simulink model "ASM_AnimationInterface"  (R2024a)
settings: Solver=ode1  StartTime=SIM.tstart.v  StopTime=SIM.tend.v  FixedStep=SIM.StepSize.v  RelTol=1e-3
PostLoadFcn:
  | , if any(exist('dsrtsu_mdlpostloadfcn', 'file') ~= 0), dsrtsu_mdlpostloadfcn('Execute', bdroot); end,
undefined symbols (not defined in the file): a0b2, b98103fe8ad365046cd0, dsmsi, MDL, SIM
libraries: simulink x22, dsmsilib x15, dsmpblib x4, ASM_Environment_lib x1
(part 6 of 7)

== system ASM_AnimationInterface/AnimationInterface/ANIMATION_INTERFACE/ASM_Vehicle/TireForceLeftFront ==
  VehicleDynamics_Animation : Inport
  Bus Selector1 : BusSelector  OutputSignals=Pos_FL_Wheel[x;y;z][m],r_Dyn_FL_Tire[m],F_FL_Tire_CoorSys_V[x;y;z][N]
  Demux : Demux  Outputs=3
  Demux2 : Demux  Outputs=3
      settings: DisplayOption=none
  Mux{,1..3} (4 alike) : Mux  Inputs=3
  Product2 : Product  SaturateOnIntegerOverflow=on  OutDataTypeStr=Inherit: Same as first input
  Sum : Sum  Inputs=+-+  InputSameDT=on  SaturateOnIntegerOverflow=on  OutDataTypeStr=Inherit: Same as first input
  Sum1 : Sum  InputSameDT=on  SaturateOnIntegerOverflow=on  OutDataTypeStr=Inherit: Same as first input
  Translation_L : Outport  VectorParamsAs1DForOutWhenUnconnected=off
  Scaling_L_x : Outport  Port=2  VectorParamsAs1DForOutWhenUnconnected=off
  Scaling_L_y : Outport  Port=3  VectorParamsAs1DForOutWhenUnconnected=off
  Scaling_L_z : Outport  Port=4  VectorParamsAs1DForOutWhenUnconnected=off
  wires:
  Mux/1 -> Translation_L/1
  [Pos_z_Offset_Arrow] -> Sum/3
  [Scaling_F_Tire] -> Product2/2
  Bus Selector1/3 -> Product2/1  "<F_FL_Tire_CoorSys_V[x;y;z][N]>"
  Bus Selector1/1 -> Demux2/1  "<Pos_FL_Wheel[x;y;z][m]>"
  Demux2/1 -> Mux/1
  Demux2/2 -> Sum1/2
  Demux2/3 -> Sum/1
  Sum/1 -> Mux/3
  Bus Selector1/2 -> Sum/2  "<r_Dyn_FL_Tire[m]>"
  VehicleDynamics_Animation/1 -> Bus Selector1/1
  Product2/1 -> Demux/1
  [Scaling_Fxy_Arrow] -> Mux3/1, Mux3/2, Mux1/1, Mux1/2, Mux2/1, Mux2/2
  Mux2/1 -> Scaling_L_z/1
  Mux1/1 -> Scaling_L_y/1
  Demux/1 -> Mux3/3
  Mux3/1 -> Scaling_L_x/1
  [Pos_y_Offset_Arrow] -> Sum1/1
  Sum1/1 -> Mux/2
  Demux/3 -> Mux2/3
  Demux/2 -> Mux1/3

== system ASM_AnimationInterface/AnimationInterface/ANIMATION_INTERFACE/ASM_Vehicle/TireForceLeftRear ==
  VehicleDynamics_Animation : Inport
  Bus Selector1 : BusSelector  OutputSignals=Pos_RL_Wheel[x;y;z][m],r_Dyn_RL_Tire[m],F_RL_Tire_CoorSys_V[x;y;z][N]
  Demux : Demux  Outputs=3
  Demux2 : Demux  Outputs=3
      settings: DisplayOption=none
  Mux{,1..3} (4 alike) : Mux  Inputs=3
  Product2 : Product  SaturateOnIntegerOverflow=on  OutDataTypeStr=Inherit: Same as first input
  Sum : Sum  Inputs=+-+  InputSameDT=on  SaturateOnIntegerOverflow=on  OutDataTypeStr=Inherit: Same as first input
  Sum1 : Sum  InputSameDT=on  SaturateOnIntegerOverflow=on  OutDataTypeStr=Inherit: Same as first input
  Translation_L : Outport  VectorParamsAs1DForOutWhenUnconnected=off
  Scaling_L_x : Outport  Port=2  VectorParamsAs1DForOutWhenUnconnected=off
  Scaling_L_y : Outport  Port=3  VectorParamsAs1DForOutWhenUnconnected=off
  Scaling_L_z : Outport  Port=4  VectorParamsAs1DForOutWhenUnconnected=off
  wires:
  Mux/1 -> Translation_L/1
  [Pos_z_Offset_Arrow] -> Sum/3
  [Scaling_F_Tire] -> Product2/2
  Bus Selector1/3 -> Product2/1  "<F_RL_Tire_CoorSys_V[x;y;z][N]>"
  Bus Selector1/1 -> Demux2/1  "<Pos_RL_Wheel[x;y;z][m]>"
  Demux2/1 -> Mux/1
  Demux2/2 -> Sum1/2
  Demux2/3 -> Sum/1
  Sum/1 -> Mux/3
  Bus Selector1/2 -> Sum/2  "<r_Dyn_RL_Tire[m]>"
  VehicleDynamics_Animation/1 -> Bus Selector1/1
  Product2/1 -> Demux/1
  Demux/3 -> Mux2/3
  [Scaling_Fxy_Arrow] -> Mux3/1, Mux3/2, Mux1/1, Mux1/2, Mux2/1, Mux2/2
  Mux2/1 -> Scaling_L_z/1
  Mux1/1 -> Scaling_L_y/1
  Demux/1 -> Mux3/3
  Mux3/1 -> Scaling_L_x/1
  [Pos_y_Offset_Arrow] -> Sum1/1
  Sum1/1 -> Mux/2
  Demux/2 -> Mux1/3

== system ASM_AnimationInterface/AnimationInterface/ANIMATION_INTERFACE/ASM_Vehicle/TireForceRightFront ==
  VehicleDynamics_Animation : Inport
  Bus Selector1 : BusSelector  OutputSignals=Pos_FR_Wheel[x;y;z][m],r_Dyn_FR_Tire[m],F_FR_Tire_CoorSys_V[x;y;z][N]
  Demux : Demux  Outputs=3
  Demux2 : Demux  Outputs=3
      settings: DisplayOption=none
  Mux{,1..3} (4 alike) : Mux  Inputs=3
  Product2 : Product  SaturateOnIntegerOverflow=on  OutDataTypeStr=Inherit: Same as first input
  Sum : Sum  Inputs=+-+  InputSameDT=on  SaturateOnIntegerOverflow=on  OutDataTypeStr=Inherit: Same as first input
  Sum1 : Sum  Inputs=-+  InputSameDT=on  SaturateOnIntegerOverflow=on  OutDataTypeStr=Inherit: Same as first input
  Translation_R : Outport  VectorParamsAs1DForOutWhenUnconnected=off
  Scaling_R_x : Outport  Port=2  VectorParamsAs1DForOutWhenUnconnected=off
  Scaling_R_y : Outport  Port=3  VectorParamsAs1DForOutWhenUnconnected=off
  Scaling_R_z : Outport  Port=4  VectorParamsAs1DForOutWhenUnconnected=off
  wires:
  Mux/1 -> Translation_R/1
  [Pos_z_Offset_Arrow] -> Sum/3
  [Scaling_F_Tire] -> Product2/2
  Bus Selector1/3 -> Product2/1  "<F_FR_Tire_CoorSys_V[x;y;z][N]>"
  Bus Selector1/1 -> Demux2/1  "<Pos_FR_Wheel[x;y;z][m]>"
  Demux2/1 -> Mux/1
  Demux2/2 -> Sum1/2
  Demux2/3 -> Sum/1
  Sum/1 -> Mux/3
  Bus Selector1/2 -> Sum/2  "<r_Dyn_FR_Tire[m]>"
  VehicleDynamics_Animation/1 -> Bus Selector1/1
  Product2/1 -> Demux/1
  Demux/3 -> Mux2/3
  [Scaling_Fxy_Arrow] -> Mux3/1, Mux3/2, Mux1/1, Mux1/2, Mux2/1, Mux2/2
  Mux2/1 -> Scaling_R_z/1
  Mux1/1 -> Scaling_R_y/1
  Demux/1 -> Mux3/3
  Mux3/1 -> Scaling_R_x/1
  [Pos_y_Offset_Arrow] -> Sum1/1
  Sum1/1 -> Mux/2
  Demux/2 -> Mux1/3

== system ASM_AnimationInterface/AnimationInterface/ANIMATION_INTERFACE/ASM_Vehicle/TireForceRightRear ==
  VehicleDynamics_Animation : Inport
  Bus Selector1 : BusSelector  OutputSignals=Pos_RR_Wheel[x;y;z][m],r_Dyn_RR_Tire[m],F_RR_Tire_CoorSys_V[x;y;z][N]
  Demux : Demux  Outputs=3
  Demux2 : Demux  Outputs=3
      settings: DisplayOption=none
  Mux{,1..3} (4 alike) : Mux  Inputs=3
  Product2 : Product  SaturateOnIntegerOverflow=on  OutDataTypeStr=Inherit: Same as first input
  Sum : Sum  Inputs=+-+  InputSameDT=on  SaturateOnIntegerOverflow=on  OutDataTypeStr=Inherit: Same as first input
  Sum1 : Sum  Inputs=-+  InputSameDT=on  SaturateOnIntegerOverflow=on  OutDataTypeStr=Inherit: Same as first input
  Translation_R : Outport  VectorParamsAs1DForOutWhenUnconnected=off
  Scaling_R_x : Outport  Port=2  VectorParamsAs1DForOutWhenUnconnected=off
  Scaling_R_y : Outport  Port=3  VectorParamsAs1DForOutWhenUnconnected=off
  Scaling_R_z : Outport  Port=4  VectorParamsAs1DForOutWhenUnconnected=off
  wires:
  Mux/1 -> Translation_R/1
  [Pos_z_Offset_Arrow] -> Sum/3
  [Scaling_F_Tire] -> Product2/2
  Bus Selector1/3 -> Product2/1  "<F_RR_Tire_CoorSys_V[x;y;z][N]>"
  Bus Selector1/1 -> Demux2/1  "<Pos_RR_Wheel[x;y;z][m]>"
  Demux2/1 -> Mux/1
  Demux2/2 -> Sum1/2
  Demux2/3 -> Sum/1
  Sum/1 -> Mux/3
  Bus Selector1/2 -> Sum/2  "<r_Dyn_RR_Tire[m]>"
  VehicleDynamics_Animation/1 -> Bus Selector1/1
  Product2/1 -> Demux/1
  Demux/3 -> Mux2/3
  [Scaling_Fxy_Arrow] -> Mux3/1, Mux3/2, Mux1/1, Mux1/2, Mux2/1, Mux2/2
  Mux2/1 -> Scaling_R_z/1
  Mux1/1 -> Scaling_R_y/1
  Demux/1 -> Mux3/3
  Mux3/1 -> Scaling_R_x/1
  [Pos_y_Offset_Arrow] -> Sum1/1
  Sum1/1 -> Mux/2
  Demux/2 -> Mux1/3

== system ASM_AnimationInterface/AnimationInterface/ANIMATION_INTERFACE/ASM_Vehicle/Wheel_FL ==
  VehicleDynamics_Animation : Inport
  Bus Selector1 : BusSelector  OutputSignals=Pos_FL_Wheel[x;y;z][m],Angle_FL_Wheel[Toe;Camber][deg],Angle_Rot_FL_Wheel[deg],r_Dyn_FL_Tire[m],Const_r_unloaded_Tire_FL[m]
  Constant1 : Constant
  Divide : Product  Inputs=*/
  Multiport Switch : MultiPortSwitch  DataPortOrder=Zero-based contiguous  Inputs=2  zeroidx=on  SaturateOnIntegerOverflow=off  InputSameDT=off
  Mux4 : Mux  Inputs=3
  Mux7 : Mux  Inputs=2
  Rotation_WheelFL : Gain  Gain=[-1 -1 1]
  Translation : Outport
  Rotation : Outport  Port=2
  Scaling : Outport  Port=3
  wires:
  Mux7/1 -> Rotation_WheelFL/1
  Rotation_WheelFL/1 -> Rotation/1
  Mux4/1 -> Scaling/1
  Bus Selector1/4 -> Divide/1  "<r_Dyn_FL_Tire[m]>"
  Bus Selector1/2 -> Mux7/1  "<Angle_FL_Wheel[Toe;Camber][deg]>"
  Bus Selector1/3 -> Mux7/2  "<Angle_Rot_FL_Wheel[deg]>"
  Bus Selector1/1 -> Translation/1  "<Pos_FL_Wheel[x;y;z][m]>"
  VehicleDynamics_Animation/1 -> Bus Selector1/1
  Constant1/1 -> Mux4/2
  [TireRadius] -> Multiport Switch/3
  Divide/1 -> Mux4/3, Mux4/1
  [Sw_TireRadius] -> Multiport Switch/1
  Bus Selector1/5 -> Multiport Switch/2  "<Const_r_unloaded_Tire_FL[m]>"
  Multiport Switch/1 -> Divide/2

== system ASM_AnimationInterface/AnimationInterface/ANIMATION_INTERFACE/ASM_Vehicle/Wheel_FR ==
  VehicleDynamics_Animation : Inport
  Bus Selector1 : BusSelector  OutputSignals=Pos_FR_Wheel[x;y;z][m],Angle_FR_Wheel[Toe;Camber][deg],Angle_Rot_FR_Wheel[deg],r_Dyn_FR_Tire[m],Const_r_unloaded_Tire_FR[m]
  Constant1 : Constant
  Divide : Product  Inputs=*/
  Multiport Switch : MultiPortSwitch  DataPortOrder=Zero-based contiguous  Inputs=2  zeroidx=on  SaturateOnIntegerOverflow=off  InputSameDT=off
  Mux4 : Mux  Inputs=3
  Mux7 : Mux  Inputs=2
  Rotation_WheelFR : Gain  Gain=[1 1 1]
  Translation : Outport
  Rotation : Outport  Port=2
  Scaling : Outport  Port=3
  wires:
  Divide/1 -> Mux4/1, Mux4/3
  Constant1/1 -> Mux4/2
  VehicleDynamics_Animation/1 -> Bus Selector1/1
  Bus Selector1/1 -> Translation/1  "<Pos_FR_Wheel[x;y;z][m]>"
  Bus Selector1/3 -> Mux7/2  "<Angle_Rot_FR_Wheel[deg]>"
  Bus Selector1/2 -> Mux7/1  "<Angle_FR_Wheel[Toe;Camber][deg]>"
  Bus Selector1/4 -> Divide/1  "<r_Dyn_FR_Tire[m]>"
  Mux4/1 -> Scaling/1
  Rotation_WheelFR/1 -> Rotation/1
  Mux7/1 -> Rotation_WheelFR/1
  Multiport Switch/1 -> Divide/2
  [TireRadius] -> Multiport Switch/3
  Bus Selector1/5 -> Multiport Switch/2  "<Const_r_unloaded_Tire_FR[m]>"
  [Sw_TireRadius] -> Multiport Switch/1

== system ASM_AnimationInterface/AnimationInterface/ANIMATION_INTERFACE/ASM_Vehicle/Wheel_RL ==
  VehicleDynamics_Animation : Inport
  Bus Selector1 : BusSelector  OutputSignals=Pos_RL_Wheel[x;y;z][m],Angle_RL_Wheel[Toe;Camber][deg],Angle_Rot_RL_Wheel[deg],r_Dyn_RL_Tire[m],Const_r_unloaded_Tire_RL[m]
  Constant1 : Constant
  Divide : Product  Inputs=*/
  Multiport Switch : MultiPortSwitch  DataPortOrder=Zero-based contiguous  Inputs=2  zeroidx=on  SaturateOnIntegerOverflow=off  InputSameDT=off
  Mux4 : Mux  Inputs=3
  Mux7 : Mux  Inputs=2
  Rotation_WheelRL : Gain  Gain=[-1 -1 1]
  Translation : Outport
  Rotation : Outport  Port=2
  Scaling : Outport  Port=3
  wires:
  Divide/1 -> Mux4/1, Mux4/3
  Constant1/1 -> Mux4/2
  VehicleDynamics_Animation/1 -> Bus Selector1/1
  Bus Selector1/1 -> Translation/1  "<Pos_RL_Wheel[x;y;z][m]>"
  Bus Selector1/3 -> Mux7/2  "<Angle_Rot_RL_Wheel[deg]>"
  Bus Selector1/2 -> Mux7/1  "<Angle_RL_Wheel[Toe;Camber][deg]>"
  Bus Selector1/4 -> Divide/1  "<r_Dyn_RL_Tire[m]>"
  Mux4/1 -> Scaling/1
  Rotation_WheelRL/1 -> Rotation/1
  Mux7/1 -> Rotation_WheelRL/1
  Multiport Switch/1 -> Divide/2
  [TireRadius] -> Multiport Switch/3
  Bus Selector1/5 -> Multiport Switch/2  "<Const_r_unloaded_Tire_RL[m]>"
  [Sw_TireRadius] -> Multiport Switch/1

== system ASM_AnimationInterface/AnimationInterface/ANIMATION_INTERFACE/ASM_Vehicle/Wheel_RR ==
  VehicleDynamics_Animation : Inport
  Bus Selector5 : BusSelector  OutputSignals=Pos_RR_Wheel[x;y;z][m],Angle_RR_Wheel[Toe;Camber][deg],Angle_Rot_RR_Wheel[deg],r_Dyn_RR_Tire[m],Const_r_unloaded_Tire_RR[m]
  Constant1 : Constant
  Divide : Product  Inputs=*/
  Multiport Switch : MultiPortSwitch  DataPortOrder=Zero-based contiguous  Inputs=2  zeroidx=on  SaturateOnIntegerOverflow=off  InputSameDT=off
  Mux4 : Mux  Inputs=3
  Mux7 : Mux  Inputs=2
  Rotation_WheelRR : Gain  Gain=[1 1 1]
  Translation : Outport
  Rotation : Outport  Port=2
  Scaling : Outport  Port=3
  wires:
  Mux7/1 -> Rotation_WheelRR/1
  Rotation_WheelRR/1 -> Rotation/1
  Mux4/1 -> Scaling/1
  Bus Selector5/4 -> Divide/1  "<r_Dyn_RR_Tire[m]>"
  Bus Selector5/2 -> Mux7/1  "<Angle_RR_Wheel[Toe;Camber][deg]>"
  Bus Selector5/3 -> Mux7/2  "<Angle_Rot_RR_Wheel[deg]>"
  Bus Selector5/1 -> Translation/1  "<Pos_RR_Wheel[x;y;z][m]>"
  VehicleDynamics_Animation/1 -> Bus Selector5/1
  Constant1/1 -> Mux4/2
  Divide/1 -> Mux4/3, Mux4/1
  Multiport Switch/1 -> Divide/2
  [TireRadius] -> Multiport Switch/3
  Bus Selector5/5 -> Multiport Switch/2  "<Const_r_unloaded_Tire_RR[m]>"
  [Sw_TireRadius] -> Multiport Switch/1

== system ASM_AnimationInterface/AnimationInterface/ANIMATION_INTERFACE/Bounding_Boxes/BoundingBox_1 ==
  Index[] : Inport
  BoundigBoxes_Animation : Inport  Port=2
  Bus Selector : BusSelector  OutputSignals=Pos_x_CoorSysE[m],Pos_y_CoorSysE[m],Pos_z_CoorSysE[m],Angle_z_Objects_CoorSysE[deg],Angle_y_Objects_CoorSysE[deg],Angle_x_Objects_CoorSysE[deg],Length_Object[m],Width_Object[m],Height_Object[m]
  Mux : Mux  Inputs=3
  Mux1 : Mux  Inputs=3
  Mux2 : Mux  Inputs=3
  Selector{1..9} (9 alike) : Selector  IndexOptions=Index vector (port)  Indices=[1 3]  OutputSizes=1
  Pos_CoorSysE[m] : Outport  VectorParamsAs1DForOutWhenUnconnected=off
  Angle_CoorSysE[m] : Outport  Port=2  VectorParamsAs1DForOutWhenUnconnected=off
  Dimensions[m] : Outport  Port=3  VectorParamsAs1DForOutWhenUnconnected=off
  wires:
  Mux2/1 -> Dimensions[m]/1
  Selector9/1 -> Mux2/3
  Selector8/1 -> Mux2/2
  Selector6/1 -> Mux2/1
  Selector4/1 -> Mux1/1
  Selector7/1 -> Mux1/3
  Selector3/1 -> Mux/3
  Selector2/1 -> Mux/2
  Selector1/1 -> Mux/1
  Index[]/1 -> Selector1/2, Selector2/2, Selector5/2, Selector7/2, Selector6/2, Selector8/2, Selector9/2, Selector4/2, Selector3/2
  Mux/1 -> Pos_CoorSysE[m]/1
  Mux1/1 -> Angle_CoorSysE[m]/1
  Selector5/1 -> Mux1/2
  BoundigBoxes_Animation/1 -> Bus Selector/1
  Bus Selector/1 -> Selector1/1  "<Pos_x_CoorSysE[m]>"
  Bus Selector/2 -> Selector2/1  "<Pos_y_CoorSysE[m]>"
  Bus Selector/3 -> Selector3/1  "<Pos_z_CoorSysE[m]>"
  Bus Selector/4 -> Selector4/1  "<Angle_z_Objects_CoorSysE[deg]>"
  Bus Selector/5 -> Selector5/1  "<Angle_y_Objects_CoorSysE[deg]>"
  Bus Selector/6 -> Selector7/1  "<Angle_x_Objects_CoorSysE[deg]>"
  Bus Selector/7 -> Selector6/1  "<Length_Object[m]>"
  Bus Selector/8 -> Selector8/1  "<Width_Object[m]>"
  Bus Selector/9 -> Selector9/1  "<Height_Object[m]>"

== system ASM_AnimationInterface/AnimationInterface/ANIMATION_INTERFACE/Bounding_Boxes/BoundingBox_10 ==
  Index[] : Inport
  BoundigBoxes_Animation : Inport  Port=2
  Bus Selector : BusSelector  OutputSignals=Pos_x_CoorSysE[m],Pos_y_CoorSysE[m],Pos_z_CoorSysE[m],Angle_z_Objects_CoorSysE[deg],Angle_y_Objects_CoorSysE[deg],Angle_x_Objects_CoorSysE[deg],Length_Object[m],Width_Object[m],Height_Object[m]
  Mux : Mux  Inputs=3
  Mux1 : Mux  Inputs=3
  Mux2 : Mux  Inputs=3
  Selector{1..9} (9 alike) : Selector  IndexOptions=Index vector (port)  Indices=[1 3]  OutputSizes=1
  Pos_CoorSysE[m] : Outport  VectorParamsAs1DForOutWhenUnconnected=off
  Angle_CoorSysE[m] : Outport  Port=2  VectorParamsAs1DForOutWhenUnconnected=off
  Dimensions[m] : Outport  Port=3  VectorParamsAs1DForOutWhenUnconnected=off
  wires:
  Mux2/1 -> Dimensions[m]/1
  Selector9/1 -> Mux2/3
  Selector8/1 -> Mux2/2
  Selector6/1 -> Mux2/1
  Selector4/1 -> Mux1/1
  Selector7/1 -> Mux1/3
  Selector3/1 -> Mux/3
  Selector2/1 -> Mux/2
  Selector1/1 -> Mux/1
  Index[]/1 -> Selector1/2, Selector2/2, Selector5/2, Selector7/2, Selector6/2, Selector8/2, Selector9/2, Selector4/2, Selector3/2
  Mux/1 -> Pos_CoorSysE[m]/1
  Mux1/1 -> Angle_CoorSysE[m]/1
  Selector5/1 -> Mux1/2
  BoundigBoxes_Animation/1 -> Bus Selector/1
  Bus Selector/1 -> Selector1/1  "<Pos_x_CoorSysE[m]>"
  Bus Selector/2 -> Selector2/1  "<Pos_y_CoorSysE[m]>"
  Bus Selector/3 -> Selector3/1  "<Pos_z_CoorSysE[m]>"
  Bus Selector/4 -> Selector4/1  "<Angle_z_Objects_CoorSysE[deg]>"
  Bus Selector/5 -> Selector5/1  "<Angle_y_Objects_CoorSysE[deg]>"
  Bus Selector/6 -> Selector7/1  "<Angle_x_Objects_CoorSysE[deg]>"
  Bus Selector/7 -> Selector6/1  "<Length_Object[m]>"
  Bus Selector/8 -> Selector8/1  "<Width_Object[m]>"
  Bus Selector/9 -> Selector9/1  "<Height_Object[m]>"

== system ASM_AnimationInterface/AnimationInterface/ANIMATION_INTERFACE/Bounding_Boxes/BoundingBox_2 ==
  Index[] : Inport
  BoundigBoxes_Animation : Inport  Port=2
  Bus Selector : BusSelector  OutputSignals=Pos_x_CoorSysE[m],Pos_y_CoorSysE[m],Pos_z_CoorSysE[m],Angle_z_Objects_CoorSysE[deg],Angle_y_Objects_CoorSysE[deg],Angle_x_Objects_CoorSysE[deg],Length_Object[m],Width_Object[m],Height_Object[m]
  Mux : Mux  Inputs=3
  Mux1 : Mux  Inputs=3
  Mux2 : Mux  Inputs=3
  Selector{1..9} (9 alike) : Selector  IndexOptions=Index vector (port)  Indices=[1 3]  OutputSizes=1
  Pos_CoorSysE[m] : Outport  VectorParamsAs1DForOutWhenUnconnected=off
  Angle_CoorSysE[m] : Outport  Port=2  VectorParamsAs1DForOutWhenUnconnected=off
  Dimensions[m] : Outport  Port=3  VectorParamsAs1DForOutWhenUnconnected=off
  wires:
  Bus Selector/9 -> Selector9/1  "<Height_Object[m]>"
  Bus Selector/8 -> Selector8/1  "<Width_Object[m]>"
  Bus Selector/7 -> Selector6/1  "<Length_Object[m]>"
  Bus Selector/6 -> Selector7/1  "<Angle_x_Objects_CoorSysE[deg]>"
  Bus Selector/5 -> Selector5/1  "<Angle_y_Objects_CoorSysE[deg]>"
  Bus Selector/4 -> Selector4/1  "<Angle_z_Objects_CoorSysE[deg]>"
  Bus Selector/3 -> Selector3/1  "<Pos_z_CoorSysE[m]>"
  Bus Selector/2 -> Selector2/1  "<Pos_y_CoorSysE[m]>"
  Bus Selector/1 -> Selector1/1  "<Pos_x_CoorSysE[m]>"
  BoundigBoxes_Animation/1 -> Bus Selector/1
  Selector5/1 -> Mux1/2
  Mux1/1 -> Angle_CoorSysE[m]/1
  Mux/1 -> Pos_CoorSysE[m]/1
  Index[]/1 -> Selector3/2, Selector4/2, Selector9/2, Selector8/2, Selector6/2, Selector7/2, Selector5/2, Selector2/2, Selector1/2
  Selector1/1 -> Mux/1
  Selector2/1 -> Mux/2
  Selector3/1 -> Mux/3
  Selector7/1 -> Mux1/3
  Selector4/1 -> Mux1/1
  Selector6/1 -> Mux2/1
  Selector8/1 -> Mux2/2
  Selector9/1 -> Mux2/3
  Mux2/1 -> Dimensions[m]/1

== system ASM_AnimationInterface/AnimationInterface/ANIMATION_INTERFACE/Bounding_Boxes/BoundingBox_3 ==
  Index[] : Inport
  BoundigBoxes_Animation : Inport  Port=2
  Bus Selector : BusSelector  OutputSignals=Pos_x_CoorSysE[m],Pos_y_CoorSysE[m],Pos_z_CoorSysE[m],Angle_z_Objects_CoorSysE[deg],Angle_y_Objects_CoorSysE[deg],Angle_x_Objects_CoorSysE[deg],Length_Object[m],Width_Object[m],Height_Object[m]
  Mux : Mux  Inputs=3
  Mux1 : Mux  Inputs=3
  Mux2 : Mux  Inputs=3
  Selector{1..9} (9 alike) : Selector  IndexOptions=Index vector (port)  Indices=[1 3]  OutputSizes=1
  Pos_CoorSysE[m] : Outport  VectorParamsAs1DForOutWhenUnconnected=off
  Angle_CoorSysE[m] : Outport  Port=2  VectorParamsAs1DForOutWhenUnconnected=off
  Dimensions[m] : Outport  Port=3  VectorParamsAs1DForOutWhenUnconnected=off
  wires:
  Bus Selector/9 -> Selector9/1  "<Height_Object[m]>"
  Bus Selector/8 -> Selector8/1  "<Width_Object[m]>"
  Bus Selector/7 -> Selector6/1  "<Length_Object[m]>"
  Bus Selector/6 -> Selector7/1  "<Angle_x_Objects_CoorSysE[deg]>"
  Bus Selector/5 -> Selector5/1  "<Angle_y_Objects_CoorSysE[deg]>"
  Bus Selector/4 -> Selector4/1  "<Angle_z_Objects_CoorSysE[deg]>"
  Bus Selector/3 -> Selector3/1  "<Pos_z_CoorSysE[m]>"
  Bus Selector/2 -> Selector2/1  "<Pos_y_CoorSysE[m]>"
  Bus Selector/1 -> Selector1/1  "<Pos_x_CoorSysE[m]>"
  BoundigBoxes_Animation/1 -> Bus Selector/1
  Selector5/1 -> Mux1/2
  Mux1/1 -> Angle_CoorSysE[m]/1
  Mux/1 -> Pos_CoorSysE[m]/1
  Index[]/1 -> Selector3/2, Selector4/2, Selector9/2, Selector8/2, Selector6/2, Selector7/2, Selector5/2, Selector2/2, Selector1/2
  Selector1/1 -> Mux/1
  Selector2/1 -> Mux/2
  Selector3/1 -> Mux/3
  Selector7/1 -> Mux1/3
  Selector4/1 -> Mux1/1
  Selector6/1 -> Mux2/1
  Selector8/1 -> Mux2/2
  Selector9/1 -> Mux2/3
  Mux2/1 -> Dimensions[m]/1

== system ASM_AnimationInterface/AnimationInterface/ANIMATION_INTERFACE/Bounding_Boxes/BoundingBox_4 ==
  Index[] : Inport
  BoundigBoxes_Animation : Inport  Port=2
  Bus Selector : BusSelector  OutputSignals=Pos_x_CoorSysE[m],Pos_y_CoorSysE[m],Pos_z_CoorSysE[m],Angle_z_Objects_CoorSysE[deg],Angle_y_Objects_CoorSysE[deg],Angle_x_Objects_CoorSysE[deg],Length_Object[m],Width_Object[m],Height_Object[m]
  Mux : Mux  Inputs=3
  Mux1 : Mux  Inputs=3
  Mux2 : Mux  Inputs=3
  Selector{1..9} (9 alike) : Selector  IndexOptions=Index vector (port)  Indices=[1 3]  OutputSizes=1
  Pos_CoorSysE[m] : Outport  VectorParamsAs1DForOutWhenUnconnected=off
  Angle_CoorSysE[m] : Outport  Port=2  VectorParamsAs1DForOutWhenUnconnected=off
  Dimensions[m] : Outport  Port=3  VectorParamsAs1DForOutWhenUnconnected=off
  wires:
  Mux2/1 -> Dimensions[m]/1
  Selector9/1 -> Mux2/3
  Selector8/1 -> Mux2/2
  Selector6/1 -> Mux2/1
  Selector4/1 -> Mux1/1
  Selector7/1 -> Mux1/3
  Selector3/1 -> Mux/3
  Selector2/1 -> Mux/2
  Selector1/1 -> Mux/1
  Index[]/1 -> Selector1/2, Selector2/2, Selector5/2, Selector7/2, Selector6/2, Selector8/2, Selector9/2, Selector4/2, Selector3/2
  Mux/1 -> Pos_CoorSysE[m]/1
  Mux1/1 -> Angle_CoorSysE[m]/1
  Selector5/1 -> Mux1/2
  BoundigBoxes_Animation/1 -> Bus Selector/1
  Bus Selector/1 -> Selector1/1  "<Pos_x_CoorSysE[m]>"
  Bus Selector/2 -> Selector2/1  "<Pos_y_CoorSysE[m]>"
  Bus Selector/3 -> Selector3/1  "<Pos_z_CoorSysE[m]>"
  Bus Selector/4 -> Selector4/1  "<Angle_z_Objects_CoorSysE[deg]>"
  Bus Selector/5 -> Selector5/1  "<Angle_y_Objects_CoorSysE[deg]>"
  Bus Selector/6 -> Selector7/1  "<Angle_x_Objects_CoorSysE[deg]>"
  Bus Selector/7 -> Selector6/1  "<Length_Object[m]>"
  Bus Selector/8 -> Selector8/1  "<Width_Object[m]>"
  Bus Selector/9 -> Selector9/1  "<Height_Object[m]>"

== system ASM_AnimationInterface/AnimationInterface/ANIMATION_INTERFACE/Bounding_Boxes/BoundingBox_5 ==
  Index[] : Inport
  BoundigBoxes_Animation : Inport  Port=2
  Bus Selector : BusSelector  OutputSignals=Pos_x_CoorSysE[m],Pos_y_CoorSysE[m],Pos_z_CoorSysE[m],Angle_z_Objects_CoorSysE[deg],Angle_y_Objects_CoorSysE[deg],Angle_x_Objects_CoorSysE[deg],Length_Object[m],Width_Object[m],Height_Object[m]
  Mux : Mux  Inputs=3
  Mux1 : Mux  Inputs=3
  Mux2 : Mux  Inputs=3
  Selector{1..9} (9 alike) : Selector  IndexOptions=Index vector (port)  Indices=[1 3]  OutputSizes=1
  Pos_CoorSysE[m] : Outport  VectorParamsAs1DForOutWhenUnconnected=off
  Angle_CoorSysE[m] : Outport  Port=2  VectorParamsAs1DForOutWhenUnconnected=off
  Dimensions[m] : Outport  Port=3  VectorParamsAs1DForOutWhenUnconnected=off
  wires:
  Bus Selector/9 -> Selector9/1  "<Height_Object[m]>"
  Bus Selector/8 -> Selector8/1  "<Width_Object[m]>"
  Bus Selector/7 -> Selector6/1  "<Length_Object[m]>"
  Bus Selector/6 -> Selector7/1  "<Angle_x_Objects_CoorSysE[deg]>"
  Bus Selector/5 -> Selector5/1  "<Angle_y_Objects_CoorSysE[deg]>"
  Bus Selector/4 -> Selector4/1  "<Angle_z_Objects_CoorSysE[deg]>"
  Bus Selector/3 -> Selector3/1  "<Pos_z_CoorSysE[m]>"
  Bus Selector/2 -> Selector2/1  "<Pos_y_CoorSysE[m]>"
  Bus Selector/1 -> Selector1/1  "<Pos_x_CoorSysE[m]>"
  BoundigBoxes_Animation/1 -> Bus Selector/1
  Selector5/1 -> Mux1/2
  Mux1/1 -> Angle_CoorSysE[m]/1
  Mux/1 -> Pos_CoorSysE[m]/1
  Index[]/1 -> Selector3/2, Selector4/2, Selector9/2, Selector8/2, Selector6/2, Selector7/2, Selector5/2, Selector2/2, Selector1/2
  Selector1/1 -> Mux/1
  Selector2/1 -> Mux/2
  Selector3/1 -> Mux/3
  Selector7/1 -> Mux1/3
  Selector4/1 -> Mux1/1
  Selector6/1 -> Mux2/1
  Selector8/1 -> Mux2/2
  Selector9/1 -> Mux2/3
  Mux2/1 -> Dimensions[m]/1

== system ASM_AnimationInterface/AnimationInterface/ANIMATION_INTERFACE/Bounding_Boxes/BoundingBox_6 ==
  Index[] : Inport
  BoundigBoxes_Animation : Inport  Port=2
  Bus Selector : BusSelector  OutputSignals=Pos_x_CoorSysE[m],Pos_y_CoorSysE[m],Pos_z_CoorSysE[m],Angle_z_Objects_CoorSysE[deg],Angle_y_Objects_CoorSysE[deg],Angle_x_Objects_CoorSysE[deg],Length_Object[m],Width_Object[m],Height_Object[m]
  Mux : Mux  Inputs=3
  Mux1 : Mux  Inputs=3
  Mux2 : Mux  Inputs=3
  Selector{1..9} (9 alike) : Selector  IndexOptions=Index vector (port)  Indices=[1 3]  OutputSizes=1
  Pos_CoorSysE[m] : Outport  VectorParamsAs1DForOutWhenUnconnected=off
  Angle_CoorSysE[m] : Outport  Port=2  VectorParamsAs1DForOutWhenUnconnected=off
  Dimensions[m] : Outport  Port=3  VectorParamsAs1DForOutWhenUnconnected=off
  wires:
  Mux2/1 -> Dimensions[m]/1
  Selector9/1 -> Mux2/3
  Selector8/1 -> Mux2/2
  Selector6/1 -> Mux2/1
  Selector4/1 -> Mux1/1
  Selector7/1 -> Mux1/3
  Selector3/1 -> Mux/3
  Selector2/1 -> Mux/2
  Selector1/1 -> Mux/1
  Index[]/1 -> Selector1/2, Selector2/2, Selector5/2, Selector7/2, Selector6/2, Selector8/2, Selector9/2, Selector4/2, Selector3/2
  Mux/1 -> Pos_CoorSysE[m]/1
  Mux1/1 -> Angle_CoorSysE[m]/1
  Selector5/1 -> Mux1/2
  BoundigBoxes_Animation/1 -> Bus Selector/1
  Bus Selector/1 -> Selector1/1  "<Pos_x_CoorSysE[m]>"
  Bus Selector/2 -> Selector2/1  "<Pos_y_CoorSysE[m]>"
  Bus Selector/3 -> Selector3/1  "<Pos_z_CoorSysE[m]>"
  Bus Selector/4 -> Selector4/1  "<Angle_z_Objects_CoorSysE[deg]>"
  Bus Selector/5 -> Selector5/1  "<Angle_y_Objects_CoorSysE[deg]>"
  Bus Selector/6 -> Selector7/1  "<Angle_x_Objects_CoorSysE[deg]>"
  Bus Selector/7 -> Selector6/1  "<Length_Object[m]>"
  Bus Selector/8 -> Selector8/1  "<Width_Object[m]>"
  Bus Selector/9 -> Selector9/1  "<Height_Object[m]>"

== system ASM_AnimationInterface/AnimationInterface/ANIMATION_INTERFACE/Bounding_Boxes/BoundingBox_7 ==
  Index[] : Inport
  BoundigBoxes_Animation : Inport  Port=2
  Bus Selector : BusSelector  OutputSignals=Pos_x_CoorSysE[m],Pos_y_CoorSysE[m],Pos_z_CoorSysE[m],Angle_z_Objects_CoorSysE[deg],Angle_y_Objects_CoorSysE[deg],Angle_x_Objects_CoorSysE[deg],Length_Object[m],Width_Object[m],Height_Object[m]
  Mux : Mux  Inputs=3
  Mux1 : Mux  Inputs=3
  Mux2 : Mux  Inputs=3
  Selector{1..9} (9 alike) : Selector  IndexOptions=Index vector (port)  Indices=[1 3]  OutputSizes=1
  Pos_CoorSysE[m] : Outport  VectorParamsAs1DForOutWhenUnconnected=off
  Angle_CoorSysE[m] : Outport  Port=2  VectorParamsAs1DForOutWhenUnconnected=off
  Dimensions[m] : Outport  Port=3  VectorParamsAs1DForOutWhenUnconnected=off
  wires:
  Mux2/1 -> Dimensions[m]/1
  Selector9/1 -> Mux2/3
  Selector8/1 -> Mux2/2
  Selector6/1 -> Mux2/1
  Selector4/1 -> Mux1/1
  Selector7/1 -> Mux1/3
  Selector3/1 -> Mux/3
  Selector2/1 -> Mux/2
  Selector1/1 -> Mux/1
  Index[]/1 -> Selector1/2, Selector2/2, Selector5/2, Selector7/2, Selector6/2, Selector8/2, Selector9/2, Selector4/2, Selector3/2
  Mux/1 -> Pos_CoorSysE[m]/1
  Mux1/1 -> Angle_CoorSysE[m]/1
  Selector5/1 -> Mux1/2
  BoundigBoxes_Animation/1 -> Bus Selector/1
  Bus Selector/1 -> Selector1/1  "<Pos_x_CoorSysE[m]>"
  Bus Selector/2 -> Selector2/1  "<Pos_y_CoorSysE[m]>"
  Bus Selector/3 -> Selector3/1  "<Pos_z_CoorSysE[m]>"
  Bus Selector/4 -> Selector4/1  "<Angle_z_Objects_CoorSysE[deg]>"
  Bus Selector/5 -> Selector5/1  "<Angle_y_Objects_CoorSysE[deg]>"
  Bus Selector/6 -> Selector7/1  "<Angle_x_Objects_CoorSysE[deg]>"
  Bus Selector/7 -> Selector6/1  "<Length_Object[m]>"
  Bus Selector/8 -> Selector8/1  "<Width_Object[m]>"
  Bus Selector/9 -> Selector9/1  "<Height_Object[m]>"

== system ASM_AnimationInterface/AnimationInterface/ANIMATION_INTERFACE/Bounding_Boxes/BoundingBox_8 ==
  Index[] : Inport
  BoundigBoxes_Animation : Inport  Port=2
  Bus Selector : BusSelector  OutputSignals=Pos_x_CoorSysE[m],Pos_y_CoorSysE[m],Pos_z_CoorSysE[m],Angle_z_Objects_CoorSysE[deg],Angle_y_Objects_CoorSysE[deg],Angle_x_Objects_CoorSysE[deg],Length_Object[m],Width_Object[m],Height_Object[m]
  Mux : Mux  Inputs=3
  Mux1 : Mux  Inputs=3
  Mux2 : Mux  Inputs=3
  Selector{1..9} (9 alike) : Selector  IndexOptions=Index vector (port)  Indices=[1 3]  OutputSizes=1
  Pos_CoorSysE[m] : Outport  VectorParamsAs1DForOutWhenUnconnected=off
  Angle_CoorSysE[m] : Outport  Port=2  VectorParamsAs1DForOutWhenUnconnected=off
  Dimensions[m] : Outport  Port=3  VectorParamsAs1DForOutWhenUnconnected=off
  wires:
  Bus Selector/9 -> Selector9/1  "<Height_Object[m]>"
  Bus Selector/8 -> Selector8/1  "<Width_Object[m]>"
  Bus Selector/7 -> Selector6/1  "<Length_Object[m]>"
  Bus Selector/6 -> Selector7/1  "<Angle_x_Objects_CoorSysE[deg]>"
  Bus Selector/5 -> Selector5/1  "<Angle_y_Objects_CoorSysE[deg]>"
  Bus Selector/4 -> Selector4/1  "<Angle_z_Objects_CoorSysE[deg]>"
  Bus Selector/3 -> Selector3/1  "<Pos_z_CoorSysE[m]>"
  Bus Selector/2 -> Selector2/1  "<Pos_y_CoorSysE[m]>"
  Bus Selector/1 -> Selector1/1  "<Pos_x_CoorSysE[m]>"
  BoundigBoxes_Animation/1 -> Bus Selector/1
  Selector5/1 -> Mux1/2
  Mux1/1 -> Angle_CoorSysE[m]/1
  Mux/1 -> Pos_CoorSysE[m]/1
  Index[]/1 -> Selector3/2, Selector4/2, Selector9/2, Selector8/2, Selector6/2, Selector7/2, Selector5/2, Selector2/2, Selector1/2
  Selector1/1 -> Mux/1
  Selector2/1 -> Mux/2
  Selector3/1 -> Mux/3
  Selector7/1 -> Mux1/3
  Selector4/1 -> Mux1/1
  Selector6/1 -> Mux2/1
  Selector8/1 -> Mux2/2
  Selector9/1 -> Mux2/3
  Mux2/1 -> Dimensions[m]/1

== system ASM_AnimationInterface/AnimationInterface/ANIMATION_INTERFACE/Bounding_Boxes/BoundingBox_9 ==
  Index[] : Inport
  BoundigBoxes_Animation : Inport  Port=2
  Bus Selector : BusSelector  OutputSignals=Pos_x_CoorSysE[m],Pos_y_CoorSysE[m],Pos_z_CoorSysE[m],Angle_z_Objects_CoorSysE[deg],Angle_y_Objects_CoorSysE[deg],Angle_x_Objects_CoorSysE[deg],Length_Object[m],Width_Object[m],Height_Object[m]
  Mux : Mux  Inputs=3
  Mux1 : Mux  Inputs=3
  Mux2 : Mux  Inputs=3
  Selector{1..9} (9 alike) : Selector  IndexOptions=Index vector (port)  Indices=[1 3]  OutputSizes=1
  Pos_CoorSysE[m] : Outport  VectorParamsAs1DForOutWhenUnconnected=off
  Angle_CoorSysE[m] : Outport  Port=2  VectorParamsAs1DForOutWhenUnconnected=off
  Dimensions[m] : Outport  Port=3  VectorParamsAs1DForOutWhenUnconnected=off
  wires:
  Bus Selector/9 -> Selector9/1  "<Height_Object[m]>"
  Bus Selector/8 -> Selector8/1  "<Width_Object[m]>"
  Bus Selector/7 -> Selector6/1  "<Length_Object[m]>"
  Bus Selector/6 -> Selector7/1  "<Angle_x_Objects_CoorSysE[deg]>"
  Bus Selector/5 -> Selector5/1  "<Angle_y_Objects_CoorSysE[deg]>"
  Bus Selector/4 -> Selector4/1  "<Angle_z_Objects_CoorSysE[deg]>"
  Bus Selector/3 -> Selector3/1  "<Pos_z_CoorSysE[m]>"
  Bus Selector/2 -> Selector2/1  "<Pos_y_CoorSysE[m]>"
  Bus Selector/1 -> Selector1/1  "<Pos_x_CoorSysE[m]>"
  BoundigBoxes_Animation/1 -> Bus Selector/1
  Selector5/1 -> Mux1/2
  Mux1/1 -> Angle_CoorSysE[m]/1
  Mux/1 -> Pos_CoorSysE[m]/1
  Index[]/1 -> Selector3/2, Selector4/2, Selector9/2, Selector8/2, Selector6/2, Selector7/2, Selector5/2, Selector2/2, Selector1/2
  Selector1/1 -> Mux/1
  Selector2/1 -> Mux/2
  Selector3/1 -> Mux/3
  Selector7/1 -> Mux1/3
  Selector4/1 -> Mux1/1
  Selector6/1 -> Mux2/1
  Selector8/1 -> Mux2/2
  Selector9/1 -> Mux2/3
  Mux2/1 -> Dimensions[m]/1

== system ASM_AnimationInterface/AnimationInterface/ANIMATION_INTERFACE/Bounding_Boxes/EnableBoxVisualization ==
  Environment_Animation : Inport
  Bus Creator : BusCreator  Inputs=9
  Bus Selector : BusSelector  OutputSignals=Boundingbox_DetectedObjects.Pos_x_CoorSysE[m],Boundingbox_DetectedObjects.Pos_y_CoorSysE[m],Boundingbox_DetectedObjects.Pos_z_CoorSysE[m],Boundingbox_DetectedObjects.Angle_x_Objects_CoorSysE[deg],Boundingbox_DetectedObjects.Angle_y_Objects_CoorSysE[deg],Boundingbox_DetectedObjects.Angle_z_Objects_CoorSysE[deg],Boundingbox_DetectedObjects.Length_Object[m],Boundingbox_DetectedObjects.Width_Object[m],Boundingbox_DetectedObjects.Height_Object[m]
  Constant : Constant  Value=zeros(1,10)
  Enable_BoxVisualization[0|1] : Constant  Value=[1 1 1 1 1 1 1 1 1 1]
  Move_Unused_Bounding_Boxes : MATLAB Function  TreatAsAtomicUnit=on
  Multiport Switch : MultiPortSwitch  DataPortOrder=Zero-based contiguous  Inputs=2  zeroidx=on  SaturateOnIntegerOverflow=off  InputSameDT=off
  Multiport Switch1 : MultiPortSwitch  DataPortOrder=Zero-based contiguous  Inputs=2  zeroidx=on  SaturateOnIntegerOverflow=off  InputSameDT=off
  Multiport Switch2 : MultiPortSwitch  DataPortOrder=Zero-based contiguous  Inputs=2  zeroidx=on  SaturateOnIntegerOverflow=off  InputSameDT=off
  BoundigBoxes_Animation : Outport  VectorParamsAs1DForOutWhenUnconnected=off
  wires:
  Multiport Switch/1 -> Move_Unused_Bounding_Boxes/1(pos_x_in)  "Pos_x_CoorSysE[m]"
  Multiport Switch1/1 -> Move_Unused_Bounding_Boxes/2(pos_y_in)  "Pos_y_CoorSysE[m]"
  Multiport Switch2/1 -> Move_Unused_Bounding_Boxes/3(pos_z_in)  "Pos_z_CoorSysE[m]"
  Enable_BoxVisualization[0|1]/1 -> Multiport Switch2/1, Multiport Switch1/1, Multiport Switch/1
  Constant/1 -> Multiport Switch2/2, Multiport Switch1/2, Multiport Switch/2
  Environment_Animation/1 -> Bus Selector/1
  Bus Selector/1 -> Multiport Switch/3  "<Pos_x_CoorSysE[m]>"
  Bus Selector/2 -> Multiport Switch1/3  "<Pos_y_CoorSysE[m]>"
  Bus Selector/3 -> Multiport Switch2/3  "<Pos_z_CoorSysE[m]>"
  Bus Selector/4 -> Move_Unused_Bounding_Boxes/4(angle_x_in)  "<Angle_x_Objects_CoorSysE[deg]>"
  Bus Selector/5 -> Move_Unused_Bounding_Boxes/5(angle_y_in)  "<Angle_y_Objects_CoorSysE[deg]>"
  Bus Selector/6 -> Move_Unused_Bounding_Boxes/6(angle_z_in)  "<Angle_z_Objects_CoorSysE[deg]>"
  Bus Creator/1 -> BoundigBoxes_Animation/1
  Move_Unused_Bounding_Boxes/1(pos_x_out) -> Bus Creator/1  "Pos_x_CoorSysE[m]"
  Move_Unused_Bounding_Boxes/2(pos_y_out) -> Bus Creator/2  "Pos_y_CoorSysE[m]"
  Move_Unused_Bounding_Boxes/3(pos_z_out) -> Bus Creator/3  "Pos_z_CoorSysE[m]"
  Move_Unused_Bounding_Boxes/4(angle_x_out) -> Bus Creator/4  "Angle_x_Objects_CoorSysE[deg]"
  Move_Unused_Bounding_Boxes/5(angle_y_out) -> Bus Creator/5  "Angle_y_Objects_CoorSysE[deg]"
  Move_Unused_Bounding_Boxes/6(angle_z_out) -> Bus Creator/6  "Angle_z_Objects_CoorSysE[deg]"
  Move_Unused_Bounding_Boxes/7(length_out) -> Bus Creator/7  "Length_Object[m]"
  Move_Unused_Bounding_Boxes/8(width_out) -> Bus Creator/8  "Width_Object[m]"
  Move_Unused_Bounding_Boxes/9(height_out) -> Bus Creator/9  "Height_Object[m]"
  Bus Selector/7 -> Move_Unused_Bounding_Boxes/7(length_in)  "<Length_Object[m]>"
  Bus Selector/8 -> Move_Unused_Bounding_Boxes/8(width_in)  "<Width_Object[m]>"
  Bus Selector/9 -> Move_Unused_Bounding_Boxes/9(height_in)  "<Height_Object[m]>"

== system ASM_AnimationInterface/AnimationInterface/ANIMATION_INTERFACE/Connection_Settings/Communication_Service ==
  Tx_Length : Inport
  Tx_Data : Inport  Port=2
  ReferenceTime[s] : Inport  Port=3
  Reset[0|1] : Inport  Port=4
  Connected_ : Constant  OutDataTypeStr=Inherit: Inherit via back propagation
  Display : Display
      settings: Format=decimal (Stored Integer)
  Rx_Data_ : Constant  Value=zeros(65507,1)  OutDataTypeStr=Inherit: Inherit via back propagation
  Rx_Length_ : Constant  Value=0  OutDataTypeStr=Inherit: Inherit via back propagation
  dsmsi_communication_service_BL1 : dsmsilib/dsmsi_communication_service_BL1  TypeOfData=Animation (Topic ID 1004)  ModelStepSize=ModelStepSize  NumSamples=NumSamples  MaxMessageSize=MaxMessageSize  blockVersion=60
      settings: SourceProductName=dSPACE MSI Blockset
  Connected : Outport
  Tx_Sent_bytes : Outport  Port=2
  Rx_Length : Outport  Port=3
  Rx_Data : Outport  Port=4
  wires:
  Tx_Data/1 -> dsmsi_communication_service_BL1/2
  Tx_Length/1 -> dsmsi_communication_service_BL1/1
  dsmsi_communication_service_BL1/1 -> Display/1
  dsmsi_communication_service_BL1/2 -> Tx_Sent_bytes/1
  Connected_/1 -> Connected/1
  Rx_Length_/1 -> Rx_Length/1
  Rx_Data_/1 -> Rx_Data/1
  Reset[0|1]/1 -> dsmsi_communication_service_BL1/4
  ReferenceTime[s]/1 -> dsmsi_communication_service_BL1/3

== system ASM_AnimationInterface/AnimationInterface/ANIMATION_INTERFACE/Connection_Settings/Communication_Service_Common_Signals ==
  Environment_Animation : Inport
  Bus Selector : BusSelector  OutputSignals=ManeuverTime[s],ManeuverState[]
  Data Type Conversion : DataTypeConversion  OutDataTypeStr=uint8  SaturateOnIntegerOverflow=off  RndMeth=Floor
  Init : simulink/Logic and Bit Operations/Compare To Constant  relop===  const=2  OutDataTypeStr=boolean
  ReferenceTime[s] : Outport
  Reset[0|1] : Outport  Port=2
  wires:
  Bus Selector/1 -> ReferenceTime[s]/1  "<ManeuverTime[s]>"
  Environment_Animation/1 -> Bus Selector/1
  Init/1 -> Data Type Conversion/1
  Data Type Conversion/1 -> Reset[0|1]/1
  Bus Selector/2 -> Init/1  "<ManeuverState[]>"

== system ASM_AnimationInterface/AnimationInterface/ANIMATION_INTERFACE/Connection_Settings/Ethernet_TCP ==
  Tx_Length : Inport
  Tx_Data : Inport  Port=2
  HIL : Subsystem  Commented=on
  MultiportSwitch{,1..3} (4 alike) : MultiPortSwitch  DataPortOrder=Zero-based contiguous  Inputs=2  zeroidx=on  SaturateOnIntegerOverflow=off  InputSameDT=off
  SIL : Subsystem  Tag=AnimationInterface_SIL
  Sw_Mode[0SIL|1HIL] : Constant  Value=Sw_Mode
  Connected : Outport
  Tx_Sent_bytes : Outport  Port=2
  Rx_Length : Outport  Port=3
  Rx_Data : Outport  Port=4
  wires:
  Tx_Data/1 -> HIL/2(Tx_Data), SIL/2(Tx_Data)
  Tx_Length/1 -> HIL/1(Tx_Length), SIL/1(Tx_Length)
  SIL/1(Connected) -> MultiportSwitch/2
  HIL/1(Connected) -> MultiportSwitch/3
  SIL/2(Tx_Sent_bytes) -> MultiportSwitch1/2
  HIL/2(Tx_Sent_bytes) -> MultiportSwitch1/3
  SIL/3(Rx_Length) -> MultiportSwitch2/2
  HIL/3(Rx_Length) -> MultiportSwitch2/3
  SIL/4(Rx_Data) -> MultiportSwitch3/2
  HIL/4(Rx_Data) -> MultiportSwitch3/3
  Sw_Mode[0SIL|1HIL]/1 -> MultiportSwitch3/1, MultiportSwitch2/1, MultiportSwitch1/1, MultiportSwitch/1
  MultiportSwitch/1 -> Connected/1
  MultiportSwitch3/1 -> Rx_Data/1
  MultiportSwitch2/1 -> Rx_Length/1
  MultiportSwitch1/1 -> Tx_Sent_bytes/1

== system ASM_AnimationInterface/AnimationInterface/ANIMATION_INTERFACE/Fellows/Fellow_Rotation ==
  In : Inport
  Bus Selector : BusSelector  OutputSignals=Angle_Yaw_Fellows[deg],Angle_Pitch_Fellows[deg],Angle_Roll_Fellows[deg]
  Reshape3 : Reshape
  Transpose2 : Math  Operator=transpose
  Vector Concatenate1 : Concatenate  NumInputs=3  Mode=Multidimensional array  ConcatenateDimension=2
  Out : Outport
  wires:
  In/1 -> Bus Selector/1
  Reshape3/1 -> Out/1
  Bus Selector/1 -> Vector Concatenate1/1  "<Angle_Yaw_Fellows[deg]>"
  Vector Concatenate1/1 -> Transpose2/1
  Bus Selector/3 -> Vector Concatenate1/3  "<Angle_Roll_Fellows[deg]>"
  Bus Selector/2 -> Vector Concatenate1/2  "<Angle_Pitch_Fellows[deg]>"
  Transpose2/1 -> Reshape3/1

== system ASM_AnimationInterface/AnimationInterface/ANIMATION_INTERFACE/Fellows/Fellow_Scaling ==
  In : Inport
  Reshape4 : Reshape
  Transpose3 : Math  Operator=transpose
  Vector Concatenate2 : Concatenate  NumInputs=3  Mode=Multidimensional array  ConcatenateDimension=2
  Out : Outport
  wires:
  In/1 -> Vector Concatenate2/3, Vector Concatenate2/2, Vector Concatenate2/1
  Transpose3/1 -> Reshape4/1
  Vector Concatenate2/1 -> Transpose3/1
  Reshape4/1 -> Out/1

== system ASM_AnimationInterface/AnimationInterface/ANIMATION_INTERFACE/Fellows/Fellow_Translation ==
  In : Inport
  Bus Selector1 : BusSelector  OutputSignals=Pos_x_Fellows[m],Pos_y_Fellows[m],Pos_z_Fellows[m]
  Reshape2 : Reshape
  Transpose1 : Math  Operator=transpose
  Vector Concatenate : Concatenate  NumInputs=3  Mode=Multidimensional array  ConcatenateDimension=2
  Out : Outport
  wires:
  Vector Concatenate/1 -> Transpose1/1
  Transpose1/1 -> Reshape2/1
  Bus Selector1/1 -> Vector Concatenate/1  "<Pos_x_Fellows[m]>"
  Bus Selector1/2 -> Vector Concatenate/2  "<Pos_y_Fellows[m]>"
  Bus Selector1/3 -> Vector Concatenate/3  "<Pos_z_Fellows[m]>"
  Reshape2/1 -> Out/1
  In/1 -> Bus Selector1/1

== system ASM_AnimationInterface/AnimationInterface/ANIMATION_INTERFACE/Lane_Sensor/Sensor_L_Rotation ==
  Sw_Pitch_Angle_Offset : Inport
  In : Inport  Port=2
  Constant1 : Constant  Value=90
  Constant2 : Constant  Value=0
  Constant3 : Constant  Value=0
  Multiport Switch : MultiPortSwitch  DataPortOrder=Zero-based contiguous  Inputs=2  zeroidx=on  SaturateOnIntegerOverflow=off  InputSameDT=off
  Mux3 : Mux  Inputs=3
  Selector : Selector  IndexOptions=Index vector (dialog)  Indices=[1]  OutputSizes=1
  Out : Outport
  wires:
  Mux3/1 -> Out/1
  Selector/1 -> Mux3/1
  In/1 -> Selector/1
  Sw_Pitch_Angle_Offset/1 -> Multiport Switch/1
  Constant2/1 -> Multiport Switch/2
  Constant1/1 -> Multiport Switch/3
  Multiport Switch/1 -> Mux3/2
  Constant3/1 -> Mux3/3

== system ASM_AnimationInterface/AnimationInterface/ANIMATION_INTERFACE/Lane_Sensor/Sensor_L_Scaling ==
  In : Inport
  CastToDouble : DataTypeConversion  OutDataTypeStr=double  SaturateOnIntegerOverflow=off  RndMeth=Floor
  Compare To Zero : simulink/Logic and Bit Operations/Compare To Zero  relop=~=  OutDataTypeStr=uint8
  Mux : Mux  Inputs=3
  Selector : Selector  IndexOptions=Index vector (dialog)  Indices=[1]  OutputSizes=1
  Out : Outport
  wires:
  Compare To Zero/1 -> CastToDouble/1
  Selector/1 -> Compare To Zero/1
  CastToDouble/1 -> Mux/3, Mux/2, Mux/1
  Mux/1 -> Out/1
  In/1 -> Selector/1

== system ASM_AnimationInterface/AnimationInterface/ANIMATION_INTERFACE/Lane_Sensor/Sensor_L_Translation ==
  In : Inport
  Bus to Vector : BusToVector
  Demux : Demux  Outputs=3
  Mux2 : Mux  Inputs=3
  Selector1 : Selector  IndexOptions=Index vector (dialog)  Indices=[1]  OutputSizes=1
  Selector2 : Selector  IndexOptions=Index vector (dialog)  Indices=[1]  OutputSizes=1
  Selector3 : Selector  IndexOptions=Index vector (dialog)  Indices=[1]  OutputSizes=1
  Out : Outport
  wires:
  Mux2/1 -> Out/1
  Selector3/1 -> Mux2/3
  Selector2/1 -> Mux2/2
  Bus to Vector/1 -> Demux/1
  Demux/3 -> Selector3/1
  Demux/1 -> Selector1/1
  Selector1/1 -> Mux2/1
  Demux/2 -> Selector2/1
  In/1 -> Bus to Vector/1

== system ASM_AnimationInterface/AnimationInterface/ANIMATION_INTERFACE/Lane_Sensor/Sensor_R_Rotation ==
  Sw_Pitch_Angle_Offset : Inport
  In : Inport  Port=2
  Constant1 : Constant  Value=90
  Constant2 : Constant  Value=0
  Constant3 : Constant  Value=0
  Multiport Switch : MultiPortSwitch  DataPortOrder=Zero-based contiguous  Inputs=2  zeroidx=on  SaturateOnIntegerOverflow=off  InputSameDT=off
  Mux3 : Mux  Inputs=3
  Selector : Selector  IndexOptions=Index vector (dialog)  Indices=[1]  OutputSizes=1
  Out : Outport
  wires:
  Sw_Pitch_Angle_Offset/1 -> Multiport Switch/1
  Constant1/1 -> Multiport Switch/3
  Constant3/1 -> Mux3/3
  In/1 -> Selector/1
  Selector/1 -> Mux3/1
  Constant2/1 -> Multiport Switch/2
  Multiport Switch/1 -> Mux3/2
  Mux3/1 -> Out/1

== system ASM_AnimationInterface/AnimationInterface/ANIMATION_INTERFACE/Lane_Sensor/Sensor_R_Scaling ==
  In : Inport
  CastToDouble : DataTypeConversion  OutDataTypeStr=double  SaturateOnIntegerOverflow=off  RndMeth=Floor
  Compare To Zero : simulink/Logic and Bit Operations/Compare To Zero  relop=~=  OutDataTypeStr=uint8
  Mux : Mux  Inputs=3
  Selector : Selector  IndexOptions=Index vector (dialog)  Indices=[1]  OutputSizes=1
  Out : Outport
  wires:
  In/1 -> Selector/1
  Mux/1 -> Out/1
  CastToDouble/1 -> Mux/1, Mux/2, Mux/3
  Selector/1 -> Compare To Zero/1
  Compare To Zero/1 -> CastToDouble/1

== system ASM_AnimationInterface/AnimationInterface/ANIMATION_INTERFACE/Lane_Sensor/Sensor_R_Translation ==
  In : Inport
  Bus to Vector : BusToVector
  Demux : Demux  Outputs=3
  Mux2 : Mux  Inputs=3
  Selector1 : Selector  IndexOptions=Index vector (dialog)  Indices=[1]  OutputSizes=1
  Selector2 : Selector  IndexOptions=Index vector (dialog)  Indices=[1]  OutputSizes=1
  Selector3 : Selector  IndexOptions=Index vector (dialog)  Indices=[1]  OutputSizes=1
  Out : Outport
  wires:
  In/1 -> Bus to Vector/1
  Demux/2 -> Selector2/1
  Selector1/1 -> Mux2/1
  Demux/1 -> Selector1/1
  Demux/3 -> Selector3/1
  Bus to Vector/1 -> Demux/1
  Selector2/1 -> Mux2/2
  Selector3/1 -> Mux2/3
  Mux2/1 -> Out/1

== system ASM_AnimationInterface/AnimationInterface/ANIMATION_INTERFACE/Lane_Sensor_Dynamic_Instruments/CalcLDWState ==
  NetworkItemType[] : Inport
  Dist_L[m] : Inport  Port=2
  Dist_R[m] : Inport  Port=3
  AND : Logic  IconShape=distinctive  AllPortsSameDT=off  OutDataTypeStr=boolean
  Compare To Constant1 : simulink/Logic and Bit Operations/Compare To Constant  relop=<=  const=0.01  OutDataTypeStr=boolean
  Compare To Constant2 : simulink/Logic and Bit Operations/Compare To Constant  relop=<=  const=0.2  OutDataTypeStr=boolean
  Compare To Constant3 : simulink/Logic and Bit Operations/Compare To Constant  relop=>  const=0.01  OutDataTypeStr=boolean
  Demux : Demux  Outputs=2
  Junction : Constant  Value=0  OutDataTypeStr=Inherit: Inherit via back propagation
  JunctionType : simulink/Logic and Bit Operations/Compare To Constant  relop===  const=3  OutDataTypeStr=boolean
  Mux : Mux  Inputs=2
  One : Constant  OutDataTypeStr=Inherit: Inherit via back propagation
  Switch : Switch  Criteria=u2 ~= 0  SaturateOnIntegerOverflow=off  InputSameDT=off
  Switch1 : Switch  Criteria=u2 ~= 0  SaturateOnIntegerOverflow=off  InputSameDT=off
  Switch2 : Switch  Criteria=u2 ~= 0  SaturateOnIntegerOverflow=off  InputSameDT=off
  Three : Constant  Value=3  OutDataTypeStr=Inherit: Inherit via back propagation
  Two : Constant  Value=2  OutDataTypeStr=Inherit: Inherit via back propagation
  LDWState_L[] : Outport  VectorParamsAs1DForOutWhenUnconnected=off
  LDWState_R[] : Outport  Port=2  VectorParamsAs1DForOutWhenUnconnected=off
  wires:
  Demux/2 -> LDWState_R[]/1
  Demux/1 -> LDWState_L[]/1
  NetworkItemType[]/1 -> JunctionType/1
  Compare To Constant3/1 -> AND/1
  Compare To Constant2/1 -> AND/2
  Compare To Constant1/1 -> Switch/2
  One/1 -> Switch/1
  AND/1 -> Switch1/2
  Three/1 -> Switch1/3
  Switch1/1 -> Switch/3
  Two/1 -> Switch1/1
  Switch/1 -> Switch2/3
  Mux/1 -> Compare To Constant3/1, Compare To Constant2/1, Compare To Constant1/1
  Dist_L[m]/1 -> Mux/1
  Dist_R[m]/1 -> Mux/2
  JunctionType/1 -> Switch2/2
  Junction/1 -> Switch2/1
  Switch2/1 -> Demux/1

== system ASM_AnimationInterface/AnimationInterface/ANIMATION_INTERFACE/Sensors/Line_Sensor_Junction_Border_Points ==
  ModelSignals : Inport
  Bus Selector : BusSelector  OutputSignals=Pos_x_Junction_Border_Animation_CoorSys_E,Pos_y_Junction_Border_Animation_CoorSys_E,Pos_z_Junction_Border_Animation_CoorSys_E
  CC : Concatenate  NumInputs=3  Mode=Multidimensional array
  Reshape1 : Reshape  OutputDimensionality=Row vector (2-D)
  Reshape2 : Reshape  OutputDimensionality=Row vector (2-D)
  Reshape3 : Reshape  OutputDimensionality=Row vector (2-D)
  AnimationSignals : Outport  VectorParamsAs1DForOutWhenUnconnected=off
  wires:
  ModelSignals/1 -> Bus Selector/1
  CC/1 -> AnimationSignals/1
  Bus Selector/1 -> Reshape1/1  "<Pos_x_Junction_Border_Animation_CoorSys_E>"
  Bus Selector/2 -> Reshape2/1  "<Pos_y_Junction_Border_Animation_CoorSys_E>"
  Bus Selector/3 -> Reshape3/1  "<Pos_z_Junction_Border_Animation_CoorSys_E>"
  Reshape1/1 -> CC/1
  Reshape2/1 -> CC/2
  Reshape3/1 -> CC/3

== system ASM_AnimationInterface/AnimationInterface/ANIMATION_INTERFACE/Sensors/Line_Sensor_Junction_Shape_ContObj_Points ==
  ModelSignals : Inport
  Bus Selector : BusSelector  OutputSignals=Pos_x_Junction_Shape_ContObj_Animation_CoorSys_E,Pos_y_Junction_Shape_ContObj_Animation_CoorSys_E,Pos_z_Junction_Shape_ContObj_Animation_CoorSys_E
  CC : Concatenate  NumInputs=3  Mode=Multidimensional array
  Reshape1 : Reshape  OutputDimensionality=Row vector (2-D)
  Reshape2 : Reshape  OutputDimensionality=Row vector (2-D)
  Reshape3 : Reshape  OutputDimensionality=Row vector (2-D)
  AnimationSignals : Outport  VectorParamsAs1DForOutWhenUnconnected=off
  wires:
  ModelSignals/1 -> Bus Selector/1
  CC/1 -> AnimationSignals/1
  Bus Selector/1 -> Reshape1/1  "<Pos_x_Junction_Shape_ContObj_Animation_CoorSys_E>"
  Bus Selector/2 -> Reshape2/1  "<Pos_y_Junction_Shape_ContObj_Animation_CoorSys_E>"
  Bus Selector/3 -> Reshape3/1  "<Pos_z_Junction_Shape_ContObj_Animation_CoorSys_E>"
  Reshape1/1 -> CC/1
  Reshape2/1 -> CC/2
  Reshape3/1 -> CC/3

== system ASM_AnimationInterface/AnimationInterface/ANIMATION_INTERFACE/Sensors/Line_Sensor_Junction_Shape_Line_Points ==
  ModelSignals : Inport
  Bus Selector : BusSelector  OutputSignals=Pos_x_Junction_Shape_Line_Animation_CoorSys_E,Pos_y_Junction_Shape_Line_Animation_CoorSys_E,Pos_z_Junction_Shape_Line_Animation_CoorSys_E
  CC : Concatenate  NumInputs=3  Mode=Multidimensional array
  Reshape1 : Reshape  OutputDimensionality=Row vector (2-D)
  Reshape2 : Reshape  OutputDimensionality=Row vector (2-D)
  Reshape3 : Reshape  OutputDimensionality=Row vector (2-D)
  AnimationSignals : Outport  VectorParamsAs1DForOutWhenUnconnected=off
  wires:
  Reshape3/1 -> CC/3
  Reshape2/1 -> CC/2
  Reshape1/1 -> CC/1
  Bus Selector/3 -> Reshape3/1  "<Pos_z_Junction_Shape_Line_Animation_CoorSys_E>"
  Bus Selector/2 -> Reshape2/1  "<Pos_y_Junction_Shape_Line_Animation_CoorSys_E>"
  Bus Selector/1 -> Reshape1/1  "<Pos_x_Junction_Shape_Line_Animation_CoorSys_E>"
  CC/1 -> AnimationSignals/1
  ModelSignals/1 -> Bus Selector/1

== system ASM_AnimationInterface/AnimationInterface/ANIMATION_INTERFACE/Sensors/Line_Sensor_Road_Lane_Points ==
  ModelSignals : Inport
  Bus Selector : BusSelector  OutputSignals=Pos_x_Road_Lane_Animation_CoorSys_E,Pos_y_Road_Lane_Animation_CoorSys_E,Pos_z_Road_Lane_Animation_CoorSys_E
  CC : Concatenate  NumInputs=3  Mode=Multidimensional array
  Reshape1 : Reshape  OutputDimensionality=Row vector (2-D)
  Reshape2 : Reshape  OutputDimensionality=Row vector (2-D)
  Reshape3 : Reshape  OutputDimensionality=Row vector (2-D)
  AnimationSignals : Outport  VectorParamsAs1DForOutWhenUnconnected=off
  wires:
  Bus Selector/3 -> Reshape3/1  "<Pos_z_Road_Lane_Animation_CoorSys_E>"
  Bus Selector/2 -> Reshape2/1  "<Pos_y_Road_Lane_Animation_CoorSys_E>"
  Bus Selector/1 -> Reshape1/1  "<Pos_x_Road_Lane_Animation_CoorSys_E>"
  CC/1 -> AnimationSignals/1
  ModelSignals/1 -> Bus Selector/1
  Reshape1/1 -> CC/1
  Reshape2/1 -> CC/2
  Reshape3/1 -> CC/3
